simulink model "FMS"  (R2018b)
settings: configuration reference "fms_config" (kept outside this file)
values from neighbouring files (symbols this model uses):
  FMS_EXPORT = Simulink.Parameter(FMS_EXPORT_VALUE)    [fms_model_init.m]
  FMS_PARAM = Simulink.Parameter(FMS_PARAM_VALUE)    [fms_model_init.m]
undefined symbols (not defined in the file or in its folder): actuator_cmd, ax_cmd, ay_cmd, az_cmd, cmd_mask, ControlMode, ctrl_mode, DiscIntNeverNeededParam, FMS_Cmd, FMS_CONST, FMS_Error, home, mode, p_cmd, phi_cmd, PilotMode, psi_rate_cmd, q_cmd, r_cmd, reset, state, status, theta_cmd, throttle_cmd, timestamp, u_cmd, v_cmd, VehicleState, VehicleStatus, w_cmd, wp_consume, wp_current
libraries: simulink x123, FMT_Model_Lib x62, hdlsllib x13
(part 3 of 7)

== system FMS/FMS Commander/Commander/Arm/Assist/Stabilize/Heading Command/Controller ==
  motion_state : Inport
  In Bus Element : Inport  Port=2  PortName=FMS_In
  In Bus Element1 : Inport  Port=2  PortName=FMS_In
  Hold Control : Subsystem  TreatAsAtomicUnit=on
  Merge : Merge
  Move Control : Subsystem  TreatAsAtomicUnit=on
  Saturation : Saturate  UpperLimit=FMS_PARAM.MC_YAWRATE_LIM  LowerLimit=-FMS_PARAM.MC_YAWRATE_LIM
  Switch Case : SwitchCase  CaseConditions={MotionState.Hold, [MotionState.Brake, MotionState.Move]}  ShowDefaultCase=off
  psi_rate_cmd_radPs : Outport
  wires:
  Move Control/1(psi_rate_cmd_radPs) -> Merge/2
  Hold Control/1(psi_rate_cmd_radPs) -> Merge/1
  In Bus Element/1 -> Hold Control/1(FMS_In)
  Switch Case/2 -> Move Control/Action
  Switch Case/1 -> Hold Control/Action
  motion_state/1 -> Switch Case/1
  Saturation/1 -> psi_rate_cmd_radPs/1
  Merge/1 -> Saturation/1
  In Bus Element1/1 -> Move Control/1(FMS_In)

== system FMS/FMS Commander/Commander/Arm/Assist/Stabilize/Heading Command/Detect Movement ==
  FMS_In : Inport
  Abs : Abs
  Abs1 : Abs
  Bus Selector : BusSelector  OutputSignals=Pilot_Cmd.stick_yaw,INS_Out.r
  Compare To Constant : simulink/Logic and Bit Operations/Compare To Constant  relop=>  const=FMS_PARAM.MC_YAW_DZ  OutDataTypeStr=boolean
  Motion State : Stateflow chart  TreatAsAtomicUnit=on
  motion_state : Outport
  wires:
  FMS_In/1 -> Bus Selector/1
  Abs1/1 -> Compare To Constant/1
  Motion State/1(state) -> motion_state/1
  Compare To Constant/1 -> Motion State/1(motion_req)
  Abs/1 -> Motion State/2(speed)
  Bus Selector/1 -> Abs1/1  "<stick_yaw>"
  Bus Selector/2 -> Abs/1  "<r>"

== system FMS/FMS Commander/Commander/Arm/Auto/Mission/Mission_SubSystem/Heading Commander ==
  FMS_In : Inport
  Bus Selector : BusSelector  OutputSignals=Cmd_In.set_yaw
  Heading Control : Subsystem
  psi_err_rad : Outport
  psi_rad_cmd : Outport  Port=2
  wires:
  FMS_In/1 -> Heading Control/1(FMS_In), Bus Selector/1
  Heading Control/1(psi_rate_cmd_radPs) -> psi_rad_cmd/1
  Heading Control/2(psi_err_rad) -> psi_err_rad/1
  Bus Selector/1 -> Heading Control/2(psi_cmd_rad)  "<set_yaw>"

== system FMS/FMS Commander/Commander/Arm/Auto/Mission/Mission_SubSystem/Velocity Commander ==
  p1 : Inport
  p2 : Inport  Port=2
  p3 : Inport  Port=3
  In Bus Element3 : Inport  Port=4  PortName=FMS_In
  In Bus Element4 : Inport  Port=4  PortName=FMS_In
  In Bus Element : Inport  Port=4  PortName=FMS_In  Element=INS_Out.vn
  In Bus Element1 : Inport  Port=4  PortName=FMS_In  Element=INS_Out.ve
  In Bus Element2 : Inport  Port=4  PortName=FMS_In  Element=INS_Out.psi
  In Bus Element6 : Inport  Port=4  PortName=FMS_In  Element=Cmd_In.set_speed
  psi_err_rad : Inport  Port=5
  Abs : Abs
  Altitude Control : Subsystem
  Compare To Constant : simulink/Logic and Bit Operations/Compare To Constant  relop=<=  const=10/180*pi  OutDataTypeStr=boolean
  Compare To Zero : simulink/Logic and Bit Operations/Compare To Zero  relop===  OutDataTypeStr=boolean
  Cruise Speed : Subsystem
  Demux : Demux  Outputs=3
  Gain : Gain  Gain=FMS_PARAM.MC_L1_GAIN  OutDataTypeStr=single
  Hold Position : Subsystem
  L1 Reference WP : Subsystem
  Lateral Acceleration : Subsystem
  Lateral Acceleration To Speed : Subsystem
  Mux1 : Mux  Inputs=2
  Switch : Switch  Criteria=u2 > Threshold
  "Target Speed " : Subsystem
  ValidCounter : Subsystem
  u_cmd : Outport
  v_cmd : Outport  Port=2
  w_cmd : Outport  Port=3
  wires:
  p3/1 -> "Target Speed "/1(P3), Lateral Acceleration To Speed/2(p3), Lateral Acceleration/3(p3), L1 Reference WP/3(P3)
  In Bus Element1/1 -> Mux1/2
  Mux1/1 -> Lateral Acceleration/1(Vg)
  p2/1 -> "Target Speed "/2(P2), Lateral Acceleration To Speed/3(p2), L1 Reference WP/2(P2)
  Demux/2 -> v_cmd/1
  Demux/3 -> w_cmd/1
  Demux/1 -> u_cmd/1
  In Bus Element/1 -> Mux1/1
  L1 Reference WP/1(L1_WP) -> Lateral Acceleration/2(L1_WP)  "L1_WP"
  p1/1 -> L1 Reference WP/1(P1)
  Gain/1 -> Lateral Acceleration/4(L1), L1 Reference WP/4(L1)
  Lateral Acceleration/1(l1_a_cmd) -> Lateral Acceleration To Speed/1(l1_a)  "l1_a_cmd"
  In Bus Element2/1 -> Lateral Acceleration To Speed/4(psi)
  "Target Speed "/1(|Vg|) -> Lateral Acceleration To Speed/5(Vg)  "Vg"
  Lateral Acceleration To Speed/1(Vg_C_cmd) -> Altitude Control/2(Vg_C_cmd)
  psi_err_rad/1 -> Abs/1
  Abs/1 -> Compare To Constant/1
  In Bus Element3/1 -> Hold Position/1(FMS_In)
  Hold Position/1(vel_cmd) -> Switch/1
  Switch/1 -> Demux/1
  Altitude Control/1(vel_C_cmd) -> Switch/3
  In Bus Element4/1 -> Altitude Control/1(FMS_In)
  Compare To Constant/1 -> ValidCounter/1(in)
  ValidCounter/1(out) -> Compare To Zero/1
  Compare To Zero/1 -> Lateral Acceleration To Speed/7(rotating), "Target Speed "/4(rotating), Switch/2
  Cruise Speed/1(cruise_speed) -> Gain/1, "Target Speed "/3(cruise_speed), Lateral Acceleration To Speed/6(cruise_speed)
  In Bus Element6/1 -> Cruise Speed/1(config_speed)

== system FMS/FMS Commander/Commander/Arm/Auto/Mission/Mission_SubSystem/Way Points ==
  note: P1: path start point
      | P2: path end point
      | P3: vehicle point
  FMS_In : Inport
  Bus Selector : BusSelector  OutputSignals=INS_Out.x_R,INS_Out.y_R
  Bus Selector1 : BusSelector  OutputSignals=Cmd_In.sp_waypoint
  Bus Selector2 : BusSelector  OutputSignals=Cmd_In.cur_waypoint
  Mux : Mux  Inputs=2
  Reshape : Reshape  OutputDimensionality=Customize  OutputDimensions=[2,1]
  Reshape1 : Reshape  OutputDimensionality=Customize  OutputDimensions=[2,1]
  Reshape2 : Reshape  OutputDimensionality=Customize  OutputDimensions=[2,1]
  Selector : Selector  InputPortWidth=3  IndexOptions=Index vector (dialog)  Indices=[1 2]  OutputSizes=1
  Selector1 : Selector  InputPortWidth=3  IndexOptions=Index vector (dialog)  Indices=[1 2]  OutputSizes=1
  p1 : Outport
  p2 : Outport  Port=2
  p3 : Outport  Port=3
  wires:
  Reshape2/1 -> p3/1
  Reshape1/1 -> p1/1
  Reshape/1 -> p2/1
  Bus Selector/2 -> Mux/2  "<y_R>"
  Bus Selector/1 -> Mux/1  "<x_R>"
  Mux/1 -> Reshape2/1
  FMS_In/1 -> Bus Selector2/1, Bus Selector1/1, Bus Selector/1
  Bus Selector1/1 -> Selector/1  "<sp_waypoint>"
  Selector/1 -> Reshape/1
  Bus Selector2/1 -> Selector1/1  "<cur_waypoint>"
  Selector1/1 -> Reshape1/1

== system FMS/FMS Commander/Commander/Arm/Auto/Offboard/Acc_Command/Accel_Command ==
  FMS_In : Inport
  Bus Selector2 : BusSelector  OutputSignals=Auto_Cmd.ax_cmd,Auto_Cmd.ay_cmd,Auto_Cmd.az_cmd
  Mux1 : Mux  Inputs=3
  accel_cmd : Outport
  wires:
  Mux1/1 -> accel_cmd/1
  FMS_In/1 -> Bus Selector2/1
  Bus Selector2/2 -> Mux1/2  "<ay_cmd>"
  Bus Selector2/1 -> Mux1/1  "<ax_cmd>"
  Bus Selector2/3 -> Mux1/3  "<az_cmd>"

== system FMS/FMS Commander/Commander/Arm/Auto/Offboard/Acc_Command/Body_FRD ==
  acc_cmd_B : Inport
  acc_cmd_C : Outport
  wires:
  acc_cmd_B/1 -> acc_cmd_C/1

== system FMS/FMS Commander/Commander/Arm/Auto/Offboard/Acc_Command/Command_Mask ==
  FMS_In : Inport
  Bus Selector1 : BusSelector  OutputSignals=Auto_Cmd.cmd_mask
  Compare To Zero2 : simulink/Logic and Bit Operations/Compare To Zero  relop=>  OutDataTypeStr=boolean
  Mux : Mux  Inputs=3
  ax_cmd valid : simulink/Logic and Bit Operations/Bitwise Operator  logicop=AND  UseBitMask=on  BitMask=bin2dec('10000000000000000')  BitMaskRealWorld=Stored Integer
  ay_cmd valid : simulink/Logic and Bit Operations/Bitwise Operator  logicop=AND  UseBitMask=on  BitMask=bin2dec('100000000000000000')  BitMaskRealWorld=Stored Integer
  az_cmd valid : simulink/Logic and Bit Operations/Bitwise Operator  logicop=AND  UseBitMask=on  BitMask=bin2dec('1000000000000000000')  BitMaskRealWorld=Stored Integer
  acc_mask : Outport
  wires:
  az_cmd valid/1 -> Mux/3
  Compare To Zero2/1 -> acc_mask/1
  ax_cmd valid/1 -> Mux/1
  ay_cmd valid/1 -> Mux/2
  FMS_In/1 -> Bus Selector1/1
  Mux/1 -> Compare To Zero2/1
  Bus Selector1/1 -> az_cmd valid/1, ay_cmd valid/1, ax_cmd valid/1  "<cmd_mask>"

== system FMS/FMS Commander/Commander/Arm/Auto/Offboard/Acc_Command/Global_Local_NED ==
  psi : Inport
  acc_cmd_O : Inport  Port=2
  Multiply : Product  Multiplication=Matrix(*)
  Psi To DCM : FMT_Model_Lib/Transformation/Psi To DCM
      settings: SourceProductName=FMT Toolbox
  acc_cmd_C : Outport
  wires:
  psi/1 -> Psi To DCM/1
  Psi To DCM/1 -> Multiply/1  "M_CO"
  acc_cmd_O/1 -> Multiply/2
  Multiply/1 -> acc_cmd_C/1

== system FMS/FMS Commander/Commander/Arm/Auto/Offboard/Acc_Command/Local_FRD ==
  psi : Inport
  acc_cmd_R : Inport  Port=2
  Data Store Read : DataStoreRead  DataStoreName=home
  Multiply3 : Product  Multiplication=Matrix(*)
  Psi To DCM2 : FMT_Model_Lib/Transformation/Psi To DCM
      settings: SourceProductName=FMT Toolbox
  Selector : Selector  InputPortWidth=4  IndexOptions=Index vector (dialog)  Indices=4  OutputSizes=1
  Subtract : Sum  Inputs=+-
  acc_cmd_C : Outport
  wires:
  Psi To DCM2/1 -> Multiply3/1  "M_CR"
  Subtract/1 -> Psi To DCM2/1
  psi/1 -> Subtract/1
  acc_cmd_R/1 -> Multiply3/2
  Multiply3/1 -> acc_cmd_C/1
  Data Store Read/1 -> Selector/1
  Selector/1 -> Subtract/2

== system FMS/FMS Commander/Commander/Arm/Auto/Offboard/Command_Mask/Subsystem ==
  note: For global/local frame, if command valid either at x or y direction,
      | then both u and v command in control frame are valid.
  frame : Inport
  cmd_mask : Inport  Port=2
  Compare To Constant : simulink/Logic and Bit Operations/Compare To Constant  relop=<=  const=2  OutDataTypeStr=boolean
  Compare To Zero{1,6..8} (4 alike) : simulink/Logic and Bit Operations/Compare To Zero  relop=>  OutDataTypeStr=boolean
  Demux : Demux  Outputs=2
  Logical Operator : Logic  Operator=OR  Inputs=3  AllPortsSameDT=off  OutDataTypeStr=boolean
  Mux : Mux  Inputs=2
  Mux1 : Mux  Inputs=2
  Switch : Switch  Criteria=u2 > Threshold
  alt_z_w_cmd : simulink/Logic and Bit Operations/Bitwise Operator  logicop=AND  UseBitMask=on  BitMask=bin2dec('1001001000000000')  BitMaskRealWorld=Stored Integer
  lat_lon_cmd valid : simulink/Logic and Bit Operations/Bitwise Operator  logicop=AND  UseBitMask=on  BitMask=bin2dec('110000000000')  BitMaskRealWorld=Stored Integer
  x_u_cmd : simulink/Logic and Bit Operations/Bitwise Operator  logicop=AND  UseBitMask=on  BitMask=bin2dec('10000010000000')  BitMaskRealWorld=Stored Integer
  y_v_cmd : simulink/Logic and Bit Operations/Bitwise Operator  logicop=AND  UseBitMask=on  BitMask=bin2dec('100000100000000')  BitMaskRealWorld=Stored Integer
  u_valid : Outport
  v_valid : Outport  Port=2
  w_valid : Outport  Port=3
  wires:
  y_v_cmd/1 -> Compare To Zero7/1
  alt_z_w_cmd/1 -> Compare To Zero8/1
  cmd_mask/1 -> lat_lon_cmd valid/1, x_u_cmd/1, alt_z_w_cmd/1, y_v_cmd/1
  x_u_cmd/1 -> Compare To Zero6/1
  frame/1 -> Compare To Constant/1
  Compare To Constant/1 -> Switch/2
  Compare To Zero7/1 -> Mux1/2, Logical Operator/3
  Logical Operator/1 -> Mux/2, Mux/1
  Compare To Zero6/1 -> Mux1/1, Logical Operator/2
  Mux1/1 -> Switch/3
  Switch/1 -> Demux/1
  Demux/1 -> u_valid/1  "uvalid"
  Demux/2 -> v_valid/1  "vvalid"
  Mux/1 -> Switch/1
  Compare To Zero8/1 -> w_valid/1  "wvalid"
  lat_lon_cmd valid/1 -> Compare To Zero1/1
  Compare To Zero1/1 -> Logical Operator/1

== system FMS/FMS Commander/Commander/Arm/Auto/Offboard/Command_Mask/Subsystem1 ==
  note: For global/local frame, if command valid either at x or y direction,
      | then both u and v command in control frame are valid.
  frame : Inport
  cmd_mask : Inport  Port=2
  Compare To Constant : simulink/Logic and Bit Operations/Compare To Constant  relop=<=  const=2  OutDataTypeStr=boolean
  Compare To Zero10 : simulink/Logic and Bit Operations/Compare To Zero  relop=>  OutDataTypeStr=boolean
  Compare To Zero11 : simulink/Logic and Bit Operations/Compare To Zero  relop=>  OutDataTypeStr=boolean
  Compare To Zero9 : simulink/Logic and Bit Operations/Compare To Zero  relop=>  OutDataTypeStr=boolean
  Demux : Demux  Outputs=2
  Logical Operator : Logic  Operator=OR  AllPortsSameDT=off  OutDataTypeStr=boolean
  Mux : Mux  Inputs=2
  Mux1 : Mux  Inputs=2
  Switch : Switch  Criteria=u2 > Threshold
  ax_cmd : simulink/Logic and Bit Operations/Bitwise Operator  logicop=AND  UseBitMask=on  BitMask=bin2dec('10000000000000000')  BitMaskRealWorld=Stored Integer
  ay_cmd : simulink/Logic and Bit Operations/Bitwise Operator  logicop=AND  UseBitMask=on  BitMask=bin2dec('100000000000000000')  BitMaskRealWorld=Stored Integer
  az_cmd : simulink/Logic and Bit Operations/Bitwise Operator  logicop=AND  UseBitMask=on  BitMask=bin2dec('1000000000000000000')  BitMaskRealWorld=Stored Integer
  ax_valid : Outport
  ay_valid : Outport  Port=2
  az_valid : Outport  Port=3
  wires:
  ax_cmd/1 -> Compare To Zero9/1
  ay_cmd/1 -> Compare To Zero10/1
  Compare To Zero11/1 -> az_valid/1
  az_cmd/1 -> Compare To Zero11/1
  Mux1/1 -> Switch/3
  Mux/1 -> Switch/1
  Logical Operator/1 -> Mux/2, Mux/1
  frame/1 -> Compare To Constant/1
  Compare To Constant/1 -> Switch/2
  Compare To Zero10/1 -> Mux1/2, Logical Operator/2
  Compare To Zero9/1 -> Mux1/1, Logical Operator/1
  cmd_mask/1 -> az_cmd/1, ax_cmd/1, ay_cmd/1
  Switch/1 -> Demux/1
  Demux/1 -> ax_valid/1
  Demux/2 -> ay_valid/1

== system FMS/FMS Commander/Commander/Arm/Auto/Offboard/Heading_Command/Heading_Control ==
  FMS_In : Inport
  Bus Selector1 : BusSelector  OutputSignals=Auto_Cmd.cmd_mask
  Compare To Zero : simulink/Logic and Bit Operations/Compare To Zero  relop=>  OutDataTypeStr=boolean
  Error : Subsystem
  Gain2 : Gain  Gain=FMS_PARAM.MC_YAW_P  OutDataTypeStr=single
  Multiply2 : Product
  psi_cmd valid : simulink/Logic and Bit Operations/Bitwise Operator  logicop=AND  UseBitMask=on  BitMask=bin2dec('100000')  BitMaskRealWorld=Stored Integer
  psi_rate_cmd : Outport
  wires:
  Compare To Zero/1 -> Multiply2/2
  Multiply2/1 -> psi_rate_cmd/1
  FMS_In/1 -> Error/1(FMS_In), Bus Selector1/1
  Bus Selector1/1 -> psi_cmd valid/1  "<cmd_mask>"
  psi_cmd valid/1 -> Compare To Zero/1
  Gain2/1 -> Multiply2/1
  Error/1(psi_error) -> Gain2/1

== system FMS/FMS Commander/Commander/Arm/Auto/Offboard/Heading_Command/Psi_Rate_Command ==
  FMS_In : Inport
  Bus Selector2 : BusSelector  OutputSignals=Auto_Cmd.psi_rate_cmd,Auto_Cmd.cmd_mask
  Compare To Zero1 : simulink/Logic and Bit Operations/Compare To Zero  relop=>  OutDataTypeStr=boolean
  Multiply1 : Product
  psi_rate_cmd valid : simulink/Logic and Bit Operations/Bitwise Operator  logicop=AND  UseBitMask=on  BitMask=bin2dec('1000000')  BitMaskRealWorld=Stored Integer
  psi_rate_cmd : Outport
  wires:
  Bus Selector2/1 -> Multiply1/1  "<psi_rate_cmd>"
  Multiply1/1 -> psi_rate_cmd/1
  psi_rate_cmd valid/1 -> Compare To Zero1/1
  FMS_In/1 -> Bus Selector2/1
  Bus Selector2/2 -> psi_rate_cmd valid/1  "<cmd_mask>"
  Compare To Zero1/1 -> Multiply1/2

== system FMS/FMS Commander/Commander/Arm/Auto/Offboard/Velocity_Command/Position_Control ==
  FMS_In : Inport
  Body_FRD : Subsystem
  Bus Selector : BusSelector  OutputSignals=INS_Out.psi
  Bus Selector2 : BusSelector  OutputSignals=Auto_Cmd.frame
  Command_Mask : Subsystem
  Gain1 : Gain  Gain=FMS_PARAM.MC_XY_P  OutDataTypeStr=single
  Gain2 : Gain  Gain=FMS_PARAM.MC_Z_P  OutDataTypeStr=single
  Global_NED : Subsystem
  Index Vector : MultiPortSwitch  DataPortOrder=Zero-based contiguous  Inputs=4  zeroidx=on
  Local_FRD : Subsystem
  Local_NED : Subsystem
  Mux1 : Mux  Inputs=2
  Position_Command : Subsystem
  Position_State : Subsystem
  Selector : Selector  InputPortWidth=3  IndexOptions=Index vector (dialog)  Indices=[1 2]  OutputSizes=1
  Selector1 : Selector  InputPortWidth=3  IndexOptions=Index vector (dialog)  Indices=3  OutputSizes=1
  vel_cmd_C : Outport
  wires:
  Mux1/1 -> vel_cmd_C/1
  Selector1/1 -> Gain2/1
  Selector/1 -> Gain1/1
  Gain1/1 -> Mux1/1
  Gain2/1 -> Mux1/2
  Index Vector/1 -> Selector1/1, Selector/1
  Command_Mask/1(pos_mask) -> Local_NED/4(pos_mask), Global_NED/4(pos_mask), Local_FRD/4(pos_mask), Body_FRD/2(pos_mask)
  Body_FRD/1(pos_error_C) -> Index Vector/5
  Local_FRD/1(pos_error_C) -> Index Vector/4
  FMS_In/1 -> Position_State/1(FMS_In), Bus Selector2/1, Command_Mask/1(FMS_In), Position_Command/1(FMS_In), Bus Selector/1
  Position_Command/1(pos_cmd) -> Local_NED/3(pos_O_cmd), Global_NED/3(pos_O_cmd), Local_FRD/3(pos_R_cmd), Body_FRD/1(pos_C_cmd)
  Bus Selector2/1 -> Index Vector/1  "<frame>"
  Position_State/1(pos_est_O) -> Local_NED/2(pos_est_O), Local_FRD/2(pos_est_O), Global_NED/2(pos_est_O)
  Bus Selector/1 -> Global_NED/1(psi), Local_NED/1(psi), Local_FRD/1(psi)  "<psi>"
  Global_NED/1(pos_error_C) -> Index Vector/2
  Local_NED/1(pos_error_C) -> Index Vector/3

== system FMS/FMS Commander/Commander/Arm/Auto/Offboard/Velocity_Command/Velocity_Command ==
  FMS_In : Inport
  Body_FRD : Subsystem
  Bus Selector1 : BusSelector  OutputSignals=INS_Out.psi
  Bus Selector3 : BusSelector  OutputSignals=Auto_Cmd.frame
  Command_Mask : Subsystem
  Global_Local_NED : Subsystem
  Index Vector : MultiPortSwitch  DataPortOrder=Zero-based contiguous  Inputs=4  zeroidx=on
  Local_FRD : Subsystem
  Multiply : Product
  Velocity_Command : Subsystem
  vel_cmd_C : Outport
  wires:
  FMS_In/1 -> Bus Selector3/1, Bus Selector1/1, Velocity_Command/1(FMS_In), Command_Mask/1(FMS_In)
  Bus Selector3/1 -> Index Vector/1  "<frame>"
  Command_Mask/1(vel_mask) -> Multiply/2
  Index Vector/1 -> vel_cmd_C/1
  Global_Local_NED/1(vel_cmd_C) -> Index Vector/3, Index Vector/2
  Local_FRD/1(vel_cmd_C) -> Index Vector/4
  Body_FRD/1(vel_cmd_C) -> Index Vector/5
  Multiply/1 -> Global_Local_NED/2(vel_cmd_O), Body_FRD/1(vel_cmd_B), Local_FRD/2(vel_cmd_L)
  Bus Selector1/1 -> Local_FRD/1(psi), Global_Local_NED/1(psi)  "<psi>"
  Velocity_Command/1(vel_cmd) -> Multiply/1

== system FMS/FMS Commander/Commander/Arm/SubMode/Hold/Altitude Hold/Controller ==
  motion_state : Inport
  In Bus Element : Inport  Port=2  PortName=FMS_In
  In Bus Element1 : Inport  Port=2  PortName=FMS_In
  Brake Control : Subsystem  TreatAsAtomicUnit=on
  Hold Control : Subsystem  TreatAsAtomicUnit=on
  Merge : Merge  Inputs=3
  Move Control : Subsystem  TreatAsAtomicUnit=on
  Saturation1 : Saturate  UpperLimit=FMS_PARAM.MC_VEL_Z_LIM  LowerLimit=-FMS_PARAM.MC_VEL_Z_LIM
  Switch Case : SwitchCase  CaseConditions={MotionState.Hold, MotionState.Brake, MotionState.Move}  ShowDefaultCase=off
  w_cmd_mPs : Outport
  wires:
  Move Control/1(w_cmd_mPs) -> Merge/3
  Brake Control/1(psi_rate_cmd_radPs) -> Merge/2
  Hold Control/1(w_cmd_mPs) -> Merge/1
  In Bus Element/1 -> Hold Control/1(FMS_In)
  Switch Case/3 -> Move Control/Action
  Switch Case/2 -> Brake Control/Action
  Switch Case/1 -> Hold Control/Action
  motion_state/1 -> Switch Case/1
  Saturation1/1 -> w_cmd_mPs/1
  Merge/1 -> Saturation1/1
  In Bus Element1/1 -> Move Control/1(FMS_In)

== system FMS/FMS Commander/Commander/Arm/SubMode/Hold/Altitude Hold/Detect Movement ==
  FMS_In : Inport
  Abs : Abs
  Bus Selector : BusSelector  OutputSignals=INS_Out.vd
  Constant : Constant  Value=0  OutDataTypeStr=Inherit: Inherit via back propagation
  Motion Status : Stateflow chart  TreatAsAtomicUnit=on
  motion_state : Outport
  wires:
  FMS_In/1 -> Bus Selector/1
  Motion Status/1(state) -> motion_state/1
  Constant/1 -> Motion Status/1(motion_req)
  Abs/1 -> Motion Status/2(speed)
  Bus Selector/1 -> Abs/1  "<vd>"

== system FMS/FMS Commander/Commander/Arm/SubMode/Hold/Heading Hold/Controller ==
  motion_state : Inport
  In Bus Element : Inport  Port=2  PortName=FMS_In
  In Bus Element1 : Inport  Port=2  PortName=FMS_In
  Brake Control : Subsystem  TreatAsAtomicUnit=on
  Hold Control : Subsystem  TreatAsAtomicUnit=on
  Merge : Merge  Inputs=3
  Move Control : Subsystem  TreatAsAtomicUnit=on
  Saturation : Saturate  UpperLimit=FMS_PARAM.MC_YAWRATE_LIM  LowerLimit=-FMS_PARAM.MC_YAWRATE_LIM
  Switch Case : SwitchCase  CaseConditions={MotionState.Hold, MotionState.Brake, MotionState.Move}  ShowDefaultCase=off
  psi_rate_cmd_radPs : Outport
  wires:
  Move Control/1(psi_rate_cmd_radPs) -> Merge/3
  Brake Control/1(psi_rate_cmd_radPs) -> Merge/2
  Hold Control/1(psi_rate_cmd_radPs) -> Merge/1
  In Bus Element/1 -> Hold Control/1(FMS_In)
  Switch Case/3 -> Move Control/Action
  Switch Case/2 -> Brake Control/Action
  Switch Case/1 -> Hold Control/Action
  motion_state/1 -> Switch Case/1
  Saturation/1 -> psi_rate_cmd_radPs/1
  Merge/1 -> Saturation/1
  In Bus Element1/1 -> Move Control/1(FMS_In)

== system FMS/FMS Commander/Commander/Arm/SubMode/Hold/Heading Hold/Detect Movement ==
  FMS_In : Inport
  Abs : Abs
  Bus Selector : BusSelector  OutputSignals=INS_Out.r
  Constant : Constant  Value=0  OutDataTypeStr=Inherit: Inherit via back propagation
  Motion State : Stateflow chart  TreatAsAtomicUnit=on
  motion_state : Outport
  wires:
  FMS_In/1 -> Bus Selector/1
  Motion State/1(state) -> motion_state/1
  Constant/1 -> Motion State/1(motion_req)
  Abs/1 -> Motion State/2(speed)
  Bus Selector/1 -> Abs/1  "<r>"

== system FMS/FMS Commander/Commander/Arm/SubMode/Hold/Position Hold/Controller ==
  motion_state : Inport
  In Bus Element : Inport  Port=2  PortName=FMS_In
  In Bus Element1 : Inport  Port=2  PortName=FMS_In
  Brake Control : Subsystem  TreatAsAtomicUnit=on
  Hold Control : Subsystem  TreatAsAtomicUnit=on
  Merge : Merge  Inputs=3
  Move Control : Subsystem  TreatAsAtomicUnit=on
  Saturation1 : Saturate  UpperLimit=FMS_PARAM.MC_VEL_XY_LIM  LowerLimit=-FMS_PARAM.MC_VEL_XY_LIM
  Switch Case : SwitchCase  CaseConditions={MotionState.Hold, MotionState.Brake, MotionState.Move}  ShowDefaultCase=off
  uv_cmd_mPs : Outport
  wires:
  Move Control/1(uv_cmd_mPs) -> Merge/3
  Brake Control/1(uv_cmd_mPs) -> Merge/2
  Hold Control/1(uv_cmd_mPs) -> Merge/1
  In Bus Element/1 -> Hold Control/1(FMS_In)
  Switch Case/3 -> Move Control/Action
  Switch Case/2 -> Brake Control/Action
  Switch Case/1 -> Hold Control/Action
  motion_state/1 -> Switch Case/1
  Saturation1/1 -> uv_cmd_mPs/1
  Merge/1 -> Saturation1/1
  In Bus Element1/1 -> Move Control/1(FMS_In)

== system FMS/FMS Commander/Commander/Arm/SubMode/Hold/Position Hold/Detect Movement ==
  FMS_In : Inport
  Add : Sum
  Bus Selector1 : BusSelector  OutputSignals=INS_Out.vn,INS_Out.ve
  Constant : Constant  Value=0  OutDataTypeStr=Inherit: Inherit via back propagation
  Motion State : Stateflow chart  TreatAsAtomicUnit=on
  Sqrt : Sqrt  SaturateOnIntegerOverflow=on
  Square : Math  Operator=square  SaturateOnIntegerOverflow=on
  Square1 : Math  Operator=square  SaturateOnIntegerOverflow=on
  motion_state : Outport
  wires:
  FMS_In/1 -> Bus Selector1/1
  Add/1 -> Sqrt/1
  Square1/1 -> Add/2
  Square/1 -> Add/1
  Motion State/1(state) -> motion_state/1  "pos_ms"
  Sqrt/1 -> Motion State/2(speed)
  Bus Selector1/1 -> Square/1  "<vn>"
  Bus Selector1/2 -> Square1/1  "<ve>"
  Constant/1 -> Motion State/1(motion_req)

== system FMS/FMS Commander/Commander/Arm/SubMode/Land/Assist Land Speed/TD ==
  v : Inport
  Integrator : DiscreteIntegrator  SampleTime=-1  ICPrevOutput=DiscIntNeverNeededParam  ICPrevScaledInput=DiscIntNeverNeededParam
  Integrator1 : DiscreteIntegrator  SampleTime=-1  ICPrevOutput=DiscIntNeverNeededParam  ICPrevScaledInput=DiscIntNeverNeededParam
  Subtract : Sum  Inputs=+-
  "fhan " : Subsystem  mask{r0=9.806, h0=0.35}
      mask DialogControl ParameterGroupVar Prompt: fhan(v1,v2,r0,h0)
  v1 : Outport
  wires:
  "fhan "/1(fhan) -> Integrator/1
  Subtract/1 -> "fhan "/1(v1)
  Integrator/1 -> Integrator1/1, "fhan "/2(v2)  "v2"
  v/1 -> Subtract/2
  Integrator1/1 -> Subtract/1, v1/1

== system FMS/FMS Commander/Commander/Arm/SubMode/Land/Position Command/Position Control ==
  FMS_In : Inport
  land_xy_R : Inport  Port=2
  Bus Selector : BusSelector  OutputSignals=INS_Out.psi
  Bus_Selection : Subsystem
  Constant : Constant  Value=0  OutDataTypeStr=Inherit: Inherit via back propagation
  Gain2 : Gain  Gain=FMS_PARAM.MC_XY_P  OutDataTypeStr=single
  Multiply : Product  Multiplication=Matrix(*)
  Mux : Mux  Inputs=2
  Psi To DCM : FMT_Model_Lib/Transformation/Psi To DCM
      settings: SourceProductName=FMT Toolbox
  Selector : Selector  InputPortWidth=3  IndexOptions=Index vector (dialog)  Indices=[1 2]  OutputSizes=1
  Sum : Sum  Inputs=-+|
  uv_cmd_mPs : Outport
  wires:
  Selector/1 -> Gain2/1
  Mux/1 -> Multiply/2
  Multiply/1 -> Selector/1
  Constant/1 -> Mux/2
  FMS_In/1 -> Bus_Selection/1(FMS_In), Bus Selector/1
  land_xy_R/1 -> Sum/2  "land_xy_sp_R"
  Sum/1 -> Mux/1  "land_xy_err_R"
  Bus_Selection/1(xy_R_O_m) -> Sum/1  "land_xy_est_R"
  Bus Selector/1 -> Psi To DCM/1  "<psi>"
  Psi To DCM/1 -> Multiply/1  "M_CO"
  Gain2/1 -> uv_cmd_mPs/1

== system FMS/FMS Commander/Commander/Arm/SubMode/Return/Heading Commander/Heading Control ==
  FMS_In : Inport
  psi_cmd_rad : Inport  Port=2
  Bus Selector : BusSelector  OutputSignals=INS_Out.psi
  Delay : Delay  DelayLength=1  InitialConditionSource=Input port
      settings: InputPortMap=u0,p4
  Heading Control : Subsystem
  Sum : Sum  Inputs=|++
  Sum1 : Sum  Inputs=+-|
  Sum2 : Sum  Inputs=|+-
  TD : Subsystem
  psi_saturation : Subsystem
  psi_saturation1 : Subsystem
  psi_rate_cmd_radPs : Outport
  psi_err_rad : Outport  Port=2
  wires:
  psi_cmd_rad/1 -> Sum2/1, Sum1/1
  Heading Control/1(psi_rate_cmd_radPs) -> psi_rate_cmd_radPs/1
  FMS_In/1 -> Heading Control/1(FMS_In), Bus Selector/1
  TD/1(v1) -> Heading Control/2(psi_cmd_rad)
  Sum1/1 -> psi_saturation1/1(psi_in)
  Bus Selector/1 -> Sum1/2, Delay/2  "<psi>"
  psi_saturation1/1(psi_rad) -> psi_err_rad/1
  Delay/1 -> Sum2/2, TD/2(v0), Sum/2, Delay/1
  Sum2/1 -> psi_saturation/1(psi_in)
  psi_saturation/1(psi_rad) -> Sum/1
  Sum/1 -> TD/1(v)

== system FMS/FMS Commander/Commander/Arm/SubMode/Return/Heading Commander/Included Angle ==
  vec1 : Inport
  vec2 : Inport  Port=2
  2D Cross Product : FMT_Model_Lib/Math/2D Cross Product
      settings: SourceProductName=FMT Toolbox
  Acos : Trigonometry  Operator=acos
  Constant4 : Constant  OutDataTypeStr=single
  Demux : Demux  Outputs=2
  Demux1 : Demux  Outputs=2
  Dot Product : DotProduct  InputSameDT=on  OutDataTypeStr=Inherit: Inherit via internal rule
  Multiply : Product
  Mux : Mux  Inputs=2
  Mux1 : Mux  Inputs=2
  Sign1 : Signum
  Switch2 : Switch  Criteria=u2 ~= 0
  Vector Normalize : FMT_Model_Lib/Math/Vector Normalize
      settings: SourceProductName=FMT Toolbox
  Vector Normalize1 : FMT_Model_Lib/Math/Vector Normalize
      settings: SourceProductName=FMT Toolbox
  angle_rad : Outport
  wires:
  Switch2/1 -> Multiply/2
  Acos/1 -> Multiply/1
  Mux/1 -> Vector Normalize1/1
  vec2/1 -> Demux/1
  Constant4/1 -> Switch2/3
  Demux/1 -> Mux/2
  vec1/1 -> Demux1/1
  Multiply/1 -> angle_rad/1
  2D Cross Product/1 -> Sign1/1
  Vector Normalize/1 -> 2D Cross Product/2, Dot Product/1
  Demux/2 -> Mux/1
  Vector Normalize1/1 -> 2D Cross Product/1, Dot Product/2
  Sign1/1 -> Switch2/2, Switch2/1
  Demux1/2 -> Mux1/1
  Mux1/1 -> Vector Normalize/1
  Demux1/1 -> Mux1/2
  Dot Product/1 -> Acos/1

== system FMS/FMS Commander/Commander/Arm/SubMode/Return/Velocity Commander/Altitude Control ==
  FMS_In : Inport
  Vg_C_cmd : Inport  Port=2
  Bus Selector3 : BusSelector  OutputSignals=INS_Out.h_R
  Gain : Gain  Gain=FMS_PARAM.MC_Z_P
  Mux : Mux  Inputs=2
  Saturation1 : Saturate  UpperLimit=FMS_PARAM.MC_VEL_Z_LIM  LowerLimit=-FMS_PARAM.MC_VEL_Z_LIM
  Selector : Selector  InputPortWidth=3  IndexOptions=Index vector (dialog)  Indices=[1 2]  OutputSizes=1
  Sum2 : Sum  Inputs=|+-
  Target Height : Subsystem
  vel_C_cmd : Outport
  wires:
  FMS_In/1 -> Bus Selector3/1, Target Height/1(FMS_In)
  Bus Selector3/1 -> Sum2/1  "<h_R>"
  Sum2/1 -> Gain/1
  Gain/1 -> Saturation1/1
  Target Height/1(h_R_sp) -> Sum2/2  "h_R_sp"
  Vg_C_cmd/1 -> Selector/1
  Selector/1 -> Mux/1
  Saturation1/1 -> Mux/2
  Mux/1 -> vel_C_cmd/1

== system FMS/FMS Commander/Commander/Arm/SubMode/Return/Velocity Commander/Cruise Speed ==
  config_speed : Inport
  Compare To Zero : simulink/Logic and Bit Operations/Compare To Zero  relop=>  OutDataTypeStr=boolean
  Switch2 : Switch  Criteria=u2 > Threshold
  vel : Constant  Value=FMS_PARAM.MC_CRUISE_SPEED  OutDataTypeStr=single
  cruise_speed : Outport
  wires:
  config_speed/1 -> Compare To Zero/1, Switch2/1
  Compare To Zero/1 -> Switch2/2
  vel/1 -> Switch2/3  "|Vg|"
  Switch2/1 -> cruise_speed/1

== system FMS/FMS Commander/Commander/Arm/SubMode/Return/Velocity Commander/Hold Position ==
  FMS_In : Inport
  Altitude Hold : Subsystem
  Mux : Mux  Inputs=3
  Position Hold : Subsystem
  vel_cmd : Outport
  wires:
  FMS_In/1 -> Altitude Hold/1(FMS_In), Position Hold/1(FMS_In)
  Position Hold/2(v_cmd_mPs) -> Mux/2
  Altitude Hold/1(w_cmd_mPs) -> Mux/3
  Position Hold/1(u_cmd_mPs) -> Mux/1
  Mux/1 -> vel_cmd/1

== system FMS/FMS Commander/Commander/Arm/SubMode/Return/Velocity Commander/L1 Reference WP ==
  P1 : Inport
  P2 : Inport  Port=2
  P3 : Inport  Port=3
  L1 : Inport  Port=4
  Compare To Constant : simulink/Logic and Bit Operations/Compare To Constant  relop=>=  const=0  OutDataTypeStr=boolean
  Compare To Constant1 : simulink/Logic and Bit Operations/Compare To Constant  relop=>  const=0  OutDataTypeStr=boolean
  NearbyRefWP : MATLAB Function  TreatAsAtomicUnit=on
  OutRegionRegWP : MATLAB Function  TreatAsAtomicUnit=on
  Reshape : Reshape  OutputDimensionality=Customize  OutputDimensions=[2,1]
  SearchL1RefWP : MATLAB Function  TreatAsAtomicUnit=on
  Switch : Switch  Criteria=u2 > Threshold
  Switch1 : Switch  Criteria=u2 > Threshold
  L1_WP : Outport
  wires:
  Reshape/1 -> L1_WP/1
  Compare To Constant/1 -> Switch/2
  NearbyRefWP/2(d) -> Compare To Constant1/1  "distance"
  SearchL1RefWP/2(u) -> Compare To Constant/1  "l1_u"
  Compare To Constant1/1 -> Switch1/2
  P1/1 -> SearchL1RefWP/1(P1), OutRegionRegWP/1(P1)
  P2/1 -> SearchL1RefWP/2(P2), NearbyRefWP/1(P2), OutRegionRegWP/2(P2)
  P3/1 -> NearbyRefWP/2(P3), SearchL1RefWP/3(P3), OutRegionRegWP/3(P3)
  Switch/1 -> Switch1/3
  L1/1 -> SearchL1RefWP/4(L1), NearbyRefWP/3(L1)
  OutRegionRegWP/1(P) -> Switch/3  "out_WP"
  Switch1/1 -> Reshape/1
  SearchL1RefWP/1(P) -> Switch/1  "L1_Ref_P"
  NearbyRefWP/1(P) -> Switch1/1  "NearbyWP"

== system FMS/FMS Commander/Commander/Arm/SubMode/Return/Velocity Commander/Lateral Acceleration ==
  Vg : Inport
  L1_WP : Inport  Port=2
  p3 : Inport  Port=3
  L1 : Inport  Port=4
  Constant : Constant  Value=0.5  OutDataTypeStr=Inherit: Inherit via back propagation
  Divide : Product  Inputs=*/
  Gain : Gain  Gain=2
  Included Angle : Subsystem
  Max : MinMax  Function=max  Inputs=2
  Min : MinMax  Inputs=2
  Multiply1 : Product
  Saturation : Saturate  UpperLimit=pi/2  LowerLimit=-pi/2
  Sin : Trigonometry
  Square : Math  Operator=square  SaturateOnIntegerOverflow=on
  Subtract : Sum  Inputs=+-
  Vector Modulus : FMT_Model_Lib/Math/Vector Modulus
      settings: SourceProductName=FMT Toolbox
  Vector Modulus1 : FMT_Model_Lib/Math/Vector Modulus
      settings: SourceProductName=FMT Toolbox
  Vector Normalize : FMT_Model_Lib/Math/Vector Normalize
      settings: SourceProductName=FMT Toolbox
  Vector Normalize1 : FMT_Model_Lib/Math/Vector Normalize
      settings: SourceProductName=FMT Toolbox
  l1_a_cmd : Outport
  wires:
  Saturation/1 -> Sin/1
  Included Angle/1(angle_rad) -> Saturation/1  "L1_alpha"
  Vector Modulus/1 -> Square/1
  Subtract/1 -> Vector Modulus1/1, Vector Normalize1/1
  Gain/1 -> Multiply1/2
  L1_WP/1 -> Subtract/1
  Vector Normalize/1 -> Included Angle/1(vec1)
  Multiply1/1 -> Divide/1
  Divide/1 -> l1_a_cmd/1  "l1_a_cmd"
  Vector Normalize1/1 -> Included Angle/2(vec2)
  Square/1 -> Gain/1
  L1/1 -> Min/1
  Vg/1 -> Vector Normalize/1, Vector Modulus/1
  Sin/1 -> Multiply1/1  "sin_alpha"
  p3/1 -> Subtract/2
  Vector Modulus1/1 -> Max/1
  Constant/1 -> Max/2
  Max/1 -> Min/2
  Min/1 -> Divide/2

== system FMS/FMS Commander/Commander/Arm/SubMode/Return/Velocity Commander/Lateral Acceleration To Speed ==
  note: If included angle between initial p3p2 and current p3p2 is larger
      | than pi/2, we need reset initial p3p2 and l1_psi
  l1_a : Inport
  p3 : Inport  Port=2
  p2 : Inport  Port=3
  psi : Inport  Port=4
  Vg : Inport  Port=5
  cruise_speed : Inport  Port=6
  rotating : Inport  Port=7
  Abs : Abs
  Compare To Constant : simulink/Logic and Bit Operations/Compare To Constant  relop=>  const=pi/2  OutDataTypeStr=boolean
  Constant1 : Constant  Value=0.5  OutDataTypeStr=single
  Delay : Delay  DelayLength=1  InitialConditionSource=Input port  ExternalReset=Level
      settings: InputPortMap=u0,r5,p4
  Delay1 : Delay  DelayLength=1
  Divide1 : Product  Inputs=*/
  Ground Speed : Subsystem
  Included Angle : Subsystem
  Logical Operator : Logic  Operator=OR  AllPortsSameDT=off  OutDataTypeStr=boolean
  Multiply : Product  Multiplication=Matrix(*)
  Rotation Matrix : Subsystem
  Saturation : Saturate  UpperLimit=pi/10  LowerLimit=-pi/10
  Saturation Dynamic : simulink/Discontinuities/Saturation Dynamic  OutMin=[]  OutMax=[]  OutDataTypeStr=Inherit: Same as second input  OutDataType=fixdt(1, 16)  OutScaling=2^-10  DoSatur=off
  Sum : Sum  Inputs=|+-
  Sum1 : Sum  Inputs=+-|
  Vg_C_cmd : Outport
  wires:
  psi/1 -> Rotation Matrix/2(psi)
  Sum/1 -> Included Angle/1(vec1), Ground Speed/2(p3p2)
  l1_a/1 -> Divide1/1
  Vg/1 -> Ground Speed/1(Vg), Saturation Dynamic/2
  p3/1 -> Sum1/2, Delay/3
  Multiply/1 -> Vg_C_cmd/1
  Rotation Matrix/1(M_CO) -> Multiply/1
  Divide1/1 -> Saturation/1
  Ground Speed/1(Vg_O_cmd) -> Multiply/2  "Vg_O_cmd"
  Delay/1 -> Delay/1, Sum/2
  Saturation/1 -> Rotation Matrix/1(l1_omega)
  cruise_speed/1 -> Saturation Dynamic/1
  Sum1/1 -> Included Angle/2(vec2)
  Included Angle/1(angle_rad) -> Abs/1
  Abs/1 -> Compare To Constant/1
  rotating/1 -> Logical Operator/1
  Compare To Constant/1 -> Delay1/1
  Logical Operator/1 -> Delay/2, Rotation Matrix/3(reset)
  p2/1 -> Sum/1, Sum1/1
  Delay1/1 -> Logical Operator/2
  Saturation Dynamic/1 -> Divide1/2
  Constant1/1 -> Saturation Dynamic/3

== system FMS/FMS Commander/Commander/Arm/SubMode/Return/Velocity Commander/Target Speed  ==
  P3 : Inport
  P2 : Inport  Port=2
  cruise_speed : Inport  Port=3
  rotating : Inport  Port=4
  Acceleration_Speed : DiscreteIntegrator  ExternalReset=level  SampleTime=-1  UpperSaturationLimit=FMS_PARAM.CRUISE_SPEED  LowerSaturationLimit=0  ICPrevOutput=DiscIntNeverNeededParam  ICPrevScaledInput=DiscIntNeverNeededParam
  Constant : Constant  Value=FMS_PARAM.MC_CRUISE_ACC  OutDataTypeStr=single
  Constant1 : Constant  Value=0.5  OutDataTypeStr=single
  Constant2 : Constant  Value=0  OutDataTypeStr=single
  Gain : Gain  Gain=0.5  OutDataTypeStr=Inherit: Same as input
  L1_GAIN : Gain  Gain=FMS_PARAM.MC_L1_GAIN  OutDataTypeStr=single
  Saturation Dynamic : simulink/Discontinuities/Saturation Dynamic  OutMin=[]  OutMax=[]  OutDataTypeStr=Inherit: Same as second input  OutDataType=fixdt(1, 16)  OutScaling=2^-10  DoSatur=off
  Saturation Dynamic1 : simulink/Discontinuities/Saturation Dynamic  OutMin=[]  OutMax=[]  OutDataTypeStr=Inherit: Same as second input  OutDataType=fixdt(1, 16)  OutScaling=2^-10  DoSatur=off
  Sum : Sum  Inputs=|+-
  Sum1 : Sum  Inputs=-+|
  Sum2 : Sum  Inputs=-+|
  Switch : Switch
  Switch1 : Switch
  Vector Modulus : FMT_Model_Lib/Math/Vector Modulus
      settings: SourceProductName=FMT Toolbox
  Vg : Outport
  wires:
  Gain/1 -> Saturation Dynamic/2
  Switch/1 -> Sum1/1, Switch1/1
  Vector Modulus/1 -> Sum2/2, Gain/1
  Sum/1 -> Vector Modulus/1
  P2/1 -> Sum/2
  P3/1 -> Sum/1
  Saturation Dynamic/1 -> Switch/3
  Constant/1 -> Acceleration_Speed/1
  Saturation Dynamic1/1 -> Switch1/3, Sum1/2
  Sum1/1 -> Switch1/2
  Switch1/1 -> Vg/1
  rotating/1 -> Acceleration_Speed/2
  cruise_speed/1 -> L1_GAIN/1, Saturation Dynamic1/1, Saturation Dynamic/1, Switch/1
  Constant1/1 -> Saturation Dynamic/3
  Acceleration_Speed/1 -> Saturation Dynamic1/2
  Constant2/1 -> Saturation Dynamic1/3
  L1_GAIN/1 -> Sum2/1
  Sum2/1 -> Switch/2

== system FMS/FMS Commander/Commander/Arm/SubMode/Return/Velocity Commander/ValidCounter ==
  in : Inport
  Compare To Constant : simulink/Logic and Bit Operations/Compare To Constant  relop=>  const=3.0  OutDataTypeStr=boolean
  Discrete-Time Integrator : DiscreteIntegrator  IntegratorMethod=Accumulation: Forward Euler  SampleTime=-1  LimitOutput=on  UpperSaturationLimit=100  LowerSaturationLimit=0  ICPrevOutput=DiscIntNeverNeededParam  ICPrevScaledInput=DiscIntNeverNeededParam
  out : Outport
  wires:
  in/1 -> Discrete-Time Integrator/1
  Discrete-Time Integrator/1 -> Compare To Constant/1
  Compare To Constant/1 -> out/1

== system FMS/FMS Commander/Commander/Arm/SubMode/Takeoff/Climb Speed/TD ==
  v : Inport
  Integrator : DiscreteIntegrator  SampleTime=-1  ICPrevOutput=DiscIntNeverNeededParam  ICPrevScaledInput=DiscIntNeverNeededParam
  Integrator1 : DiscreteIntegrator  SampleTime=-1  ICPrevOutput=DiscIntNeverNeededParam  ICPrevScaledInput=DiscIntNeverNeededParam
  Subtract : Sum  Inputs=+-
  "fhan " : Subsystem  mask{r0=9.806, h0=0.35}
      mask DialogControl ParameterGroupVar Prompt: fhan(v1,v2,r0,h0)
  v1 : Outport
  wires:
  "fhan "/1(fhan) -> Integrator/1
  Subtract/1 -> "fhan "/1(v1)
  Integrator/1 -> Integrator1/1, "fhan "/2(v2)  "v2"
  v/1 -> Subtract/2
  Integrator1/1 -> Subtract/1, v1/1

== system FMS/FMS Commander/Commander/Arm/SubMode/Takeoff/Track Position/Bus_Selection ==
  FMS_In : Inport
  Bus Selector2 : BusSelector  OutputSignals=INS_Out.x_R,INS_Out.y_R
  Mux : Mux  Inputs=2
  xy_est_R : Outport
  wires:
  Bus Selector2/2 -> Mux/2  "<y_R>"
  Mux/1 -> xy_est_R/1
  Bus Selector2/1 -> Mux/1  "<x_R>"
  FMS_In/1 -> Bus Selector2/1

== system FMS/FMS Commander/Commander/Arm/SubMode/Takeoff/Track Position/Target Position ==
  FMS_In : Inport
  Bus Selector1 : BusSelector  OutputSignals=Cmd_In.sp_waypoint
  Bus Selector2 : BusSelector  OutputSignals=INS_Out.x_R,INS_Out.y_R,INS_Out.h_R
  Divide : Product  Inputs=/*
  Multiply : Product
  Mux : Mux  Inputs=3
  Reshape : Reshape  OutputDimensionality=Column vector (2-D)  OutputDimensions=[2,1]
  Saturation : Saturate  UpperLimit=1  LowerLimit=0
  Selector1 : Selector  InputPortWidth=3  IndexOptions=Index vector (dialog)  Indices=[1 2]  OutputSizes=1
  Selector2 : Selector  InputPortWidth=3  IndexOptions=Index vector (dialog)  Indices=3  OutputSizes=1
  Selector3 : Selector  InputPortWidth=3  IndexOptions=Index vector (dialog)  Indices=3  OutputSizes=1
  Selector4 : Selector  InputPortWidth=3  IndexOptions=Index vector (dialog)  Indices=[1 2]  OutputSizes=1
  Sum1 : Sum  Inputs=|+-
  Sum2 : Sum  Inputs=-+|
  Sum3 : Sum  Inputs=|+-
  Sum4 : Sum  Inputs=|++
  cur_waypoint : Delay  DelayLength=1  InitialConditionSource=Input port  InitialCondition=single([0 0])
      settings: InputPortMap=u0,p4
  xy_cmd_R : Outport
  wires:
  Bus Selector2/3 -> Mux/3, Sum2/2  "<h_R>"
  Saturation/1 -> Multiply/2
  Selector3/1 -> Sum2/1, Sum1/2
  cur_waypoint/1 -> Selector3/1, Selector4/1, cur_waypoint/1
  Sum2/1 -> Divide/2
  Selector2/1 -> Sum1/1
  Divide/1 -> Saturation/1
  FMS_In/1 -> Bus Selector2/1, Bus Selector1/1
  Sum1/1 -> Divide/1
  Bus Selector1/1 -> Selector1/1, Selector2/1  "<sp_waypoint>"
  Selector1/1 -> Sum3/1
  Selector4/1 -> Sum4/2, Sum3/2
  Sum3/1 -> Multiply/1
  Multiply/1 -> Sum4/1
  Sum4/1 -> Reshape/1
  Reshape/1 -> xy_cmd_R/1
  Mux/1 -> cur_waypoint/2
  Bus Selector2/2 -> Mux/2  "<y_R>"
  Bus Selector2/1 -> Mux/1  "<x_R>"

== system FMS/FMS Commander/Commander/Arm/Assist/Altitude/Altitude Command/Controller/Hold Control ==
  FMS_In : Inport
  Action Port : ActionPort  InitializeStates=reset  ActionType=case
  Bus_Selection : Subsystem
  Delay : Delay  DelayLength=1  InitialConditionSource=Input port
      settings: InputPortMap=u0,p4
  Gain2 : Gain  Gain=FMS_PARAM.MC_Z_P  OutDataTypeStr=single
  Sum : Sum  Inputs=-+|
  w_cmd_mPs : Outport
  wires:
  FMS_In/1 -> Bus_Selection/1(FMS_In)
  Delay/1 -> Sum/2, Delay/1  "z_cmd_R"
  Sum/1 -> Gain2/1  "z_err_R"
  Bus_Selection/1(z_R_m) -> Delay/2, Sum/1  "z_est_R"
  Gain2/1 -> w_cmd_mPs/1

== system FMS/FMS Commander/Commander/Arm/Assist/Altitude/Altitude Command/Controller/Move Control ==
  FMS_In : Inport
  Action Port : ActionPort  InitializeStates=reset  ActionType=case
  Assist Land Speed : Subsystem
  Bus Selector : BusSelector  OutputSignals=Pilot_Cmd.stick_throttle
  Bus Selector1 : BusSelector  OutputSignals=INS_Out.flag,INS_Out.h_AGL
  Compare To Constant : simulink/Logic and Bit Operations/Compare To Constant  relop=<=  const=FMS_PARAM.MC_ASSIST_LAND_H  OutDataTypeStr=boolean
  Compare To Constant1 : simulink/Logic and Bit Operations/Compare To Constant  relop=>  const=0  OutDataTypeStr=boolean
  DeadZone : Subsystem  mask{th=FMS_PARAM.MC_THROTTLE_DZ}
      mask prompts: th "Threshold"
      mask Display: disp('Dead Zone')
  Gain1 : Gain  Gain=-FMS_PARAM.MC_VEL_Z_LIM  OutDataTypeStr=single
  Logical Operator : Logic  Inputs=3  AllPortsSameDT=off  OutDataTypeStr=boolean
  Switch : Switch  Criteria=u2 > Threshold
  cmd_p valid : simulink/Logic and Bit Operations/Bitwise Operator  logicop=AND  UseBitMask=on  BitMask=bin2dec('100000000')  BitMaskRealWorld=Stored Integer
  w_cmd_mPs : Outport
  wires:
  cmd_p valid/1 -> Logical Operator/2  "h_AGL_valid"
  Compare To Constant1/1 -> Logical Operator/1
  Bus Selector1/1 -> cmd_p valid/1  "<flag>"
  Compare To Constant/1 -> Logical Operator/3
  DeadZone/1(y) -> Gain1/1
  Bus Selector1/2 -> Compare To Constant/1  "<h_AGL>"
  Bus Selector/1 -> DeadZone/1(u)  "<stick_throttle>"
  Logical Operator/1 -> Switch/2
  Gain1/1 -> Compare To Constant1/1, Assist Land Speed/1(u), Switch/3
  FMS_In/1 -> Bus Selector1/1, Bus Selector/1
  Assist Land Speed/1(y) -> Switch/1
  Switch/1 -> w_cmd_mPs/1

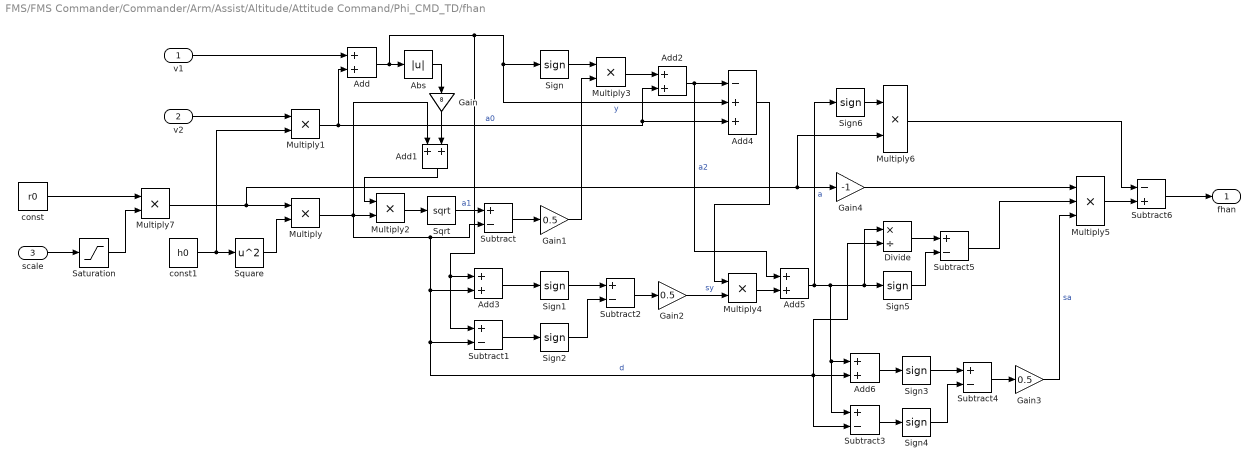
== system FMS/FMS Commander/Commander/Arm/Assist/Altitude/Attitude Command/Phi_CMD_TD/fhan  ==
  v1 : Inport
  v2 : Inport  Port=2
  scale : Inport  Port=3
  Abs : Abs
  Add{,1..3,5..6} (6 alike) : Sum  OutDataTypeStr=Inherit: Same as first input
  Add4 : Sum  Inputs=-++
  Divide : Product  Inputs=*/
  Gain : Gain  Gain=8
  Gain1 : Gain  Gain=0.5  OutDataTypeStr=Inherit: Same as input
  Gain2 : Gain  Gain=0.5  OutDataTypeStr=Inherit: Same as input
  Gain3 : Gain  Gain=0.5  OutDataTypeStr=Inherit: Same as input
  Gain4 : Gain  Gain=-1  OutDataTypeStr=Inherit: Same as input
  Multiply{,1..3} (4 alike) : Product  OutDataTypeStr=Inherit: Same as first input
  Multiply4 : Product  OutDataTypeStr=single
  Multiply5 : Product  Inputs=3
  Multiply6 : Product  OutDataTypeStr=single
  Multiply7 : Product
  Saturation : Saturate  UpperLimit=1  LowerLimit=0
  Sign{,1..6} (7 alike) : Signum
  Sqrt : Sqrt  SaturateOnIntegerOverflow=on
  Square : Math  Operator=square  SaturateOnIntegerOverflow=on
  Subtract{,1..5} (6 alike) : Sum  Inputs=+-  OutDataTypeStr=Inherit: Same as first input
  Subtract6 : Sum  Inputs=-+  OutDataTypeStr=Inherit: Same as first input
  const : Constant  Value=r0  OutDataTypeStr=single
  const1 : Constant  Value=h0  OutDataTypeStr=single
  fhan : Outport
  wires:
  v1/1 -> Add/1
  Sign/1 -> Multiply3/1
  Gain2/1 -> Multiply4/2  "sy"
  v2/1 -> Multiply1/1
  Gain3/1 -> Multiply5/3  "sa"
  Subtract/1 -> Gain1/1
  Subtract6/1 -> fhan/1
  Sign2/1 -> Subtract2/2
  Sign4/1 -> Subtract4/2
  Abs/1 -> Gain/1
  Add4/1 -> Multiply4/1
  Sign5/1 -> Subtract5/2
  Sqrt/1 -> Subtract/1  "a1"
  Subtract3/1 -> Sign4/1
  Add1/1 -> Multiply2/1
  Subtract1/1 -> Sign2/1
  Divide/1 -> Subtract5/1
  Multiply3/1 -> Add2/1
  Gain/1 -> Add1/2
  Multiply7/1 -> Multiply6/2, Gain4/1, Multiply/1
  Add3/1 -> Sign1/1
  Subtract5/1 -> Multiply5/2
  Multiply4/1 -> Add5/2
  const1/1 -> Multiply1/2, Square/1
  Add5/1 -> Sign6/1, Sign5/1, Divide/1, Subtract3/1, Add6/1  "a"
  Multiply1/1 -> Add4/3, Add2/2, Add/2  "a0"
  Add/1 -> Subtract1/1, Add3/1, Add4/2, Sign/1, Abs/1  "y"
  Subtract2/1 -> Gain2/1
  Add2/1 -> Add4/1, Add5/1  "a2"
  Subtract4/1 -> Gain3/1
  Gain4/1 -> Multiply5/1
  Multiply5/1 -> Subtract6/2
  Sign6/1 -> Multiply6/1
  Sign3/1 -> Subtract4/1
  Add6/1 -> Sign3/1
  Multiply/1 -> Subtract/2, Divide/2, Subtract3/2, Add6/2, Subtract1/2, Add3/2, Add1/1, Multiply2/2  "d"
  Multiply6/1 -> Subtract6/1
  Gain1/1 -> Multiply3/2
  Square/1 -> Multiply/2
  Multiply2/1 -> Sqrt/1
  Sign1/1 -> Subtract2/1
  scale/1 -> Saturation/1
  const/1 -> Multiply7/1
  Saturation/1 -> Multiply7/2

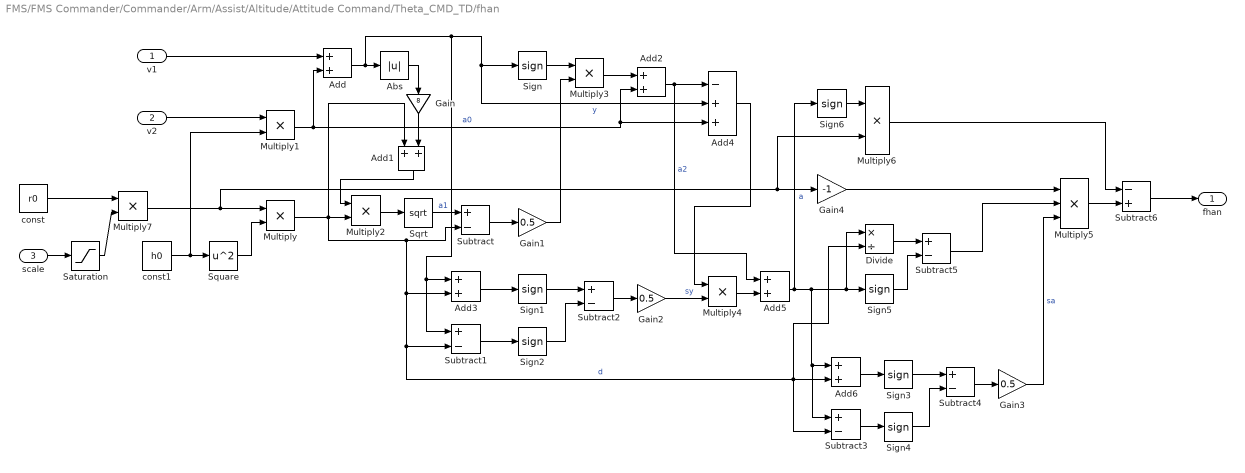
== system FMS/FMS Commander/Commander/Arm/Assist/Altitude/Attitude Command/Theta_CMD_TD/fhan  ==
  v1 : Inport
  v2 : Inport  Port=2
  scale : Inport  Port=3
  Abs : Abs
  Add{,1..3,5..6} (6 alike) : Sum  OutDataTypeStr=Inherit: Same as first input
  Add4 : Sum  Inputs=-++
  Divide : Product  Inputs=*/
  Gain : Gain  Gain=8
  Gain1 : Gain  Gain=0.5  OutDataTypeStr=Inherit: Same as input
  Gain2 : Gain  Gain=0.5  OutDataTypeStr=Inherit: Same as input
  Gain3 : Gain  Gain=0.5  OutDataTypeStr=Inherit: Same as input
  Gain4 : Gain  Gain=-1  OutDataTypeStr=Inherit: Same as input
  Multiply{,1..3} (4 alike) : Product  OutDataTypeStr=Inherit: Same as first input
  Multiply4 : Product  OutDataTypeStr=single
  Multiply5 : Product  Inputs=3
  Multiply6 : Product  OutDataTypeStr=single
  Multiply7 : Product
  Saturation : Saturate  UpperLimit=1  LowerLimit=0
  Sign{,1..6} (7 alike) : Signum
  Sqrt : Sqrt  SaturateOnIntegerOverflow=on
  Square : Math  Operator=square  SaturateOnIntegerOverflow=on
  Subtract{,1..5} (6 alike) : Sum  Inputs=+-  OutDataTypeStr=Inherit: Same as first input
  Subtract6 : Sum  Inputs=-+  OutDataTypeStr=Inherit: Same as first input
  const : Constant  Value=r0  OutDataTypeStr=single
  const1 : Constant  Value=h0  OutDataTypeStr=single
  fhan : Outport
  wires:
  v1/1 -> Add/1
  Sign/1 -> Multiply3/1
  Gain2/1 -> Multiply4/2  "sy"
  v2/1 -> Multiply1/1
  Gain3/1 -> Multiply5/3  "sa"
  Subtract/1 -> Gain1/1
  Subtract6/1 -> fhan/1
  Sign2/1 -> Subtract2/2
  Sign4/1 -> Subtract4/2
  Abs/1 -> Gain/1
  Add4/1 -> Multiply4/1
  Sign5/1 -> Subtract5/2
  Sqrt/1 -> Subtract/1  "a1"
  Subtract3/1 -> Sign4/1
  Add1/1 -> Multiply2/1
  Subtract1/1 -> Sign2/1
  Divide/1 -> Subtract5/1
  Multiply3/1 -> Add2/1
  Gain/1 -> Add1/2
  Multiply7/1 -> Multiply6/2, Gain4/1, Multiply/1
  Add3/1 -> Sign1/1
  Subtract5/1 -> Multiply5/2
  Multiply4/1 -> Add5/2
  const1/1 -> Multiply1/2, Square/1
  Add5/1 -> Sign6/1, Sign5/1, Divide/1, Subtract3/1, Add6/1  "a"
  Multiply1/1 -> Add4/3, Add2/2, Add/2  "a0"
  Add/1 -> Subtract1/1, Add3/1, Add4/2, Sign/1, Abs/1  "y"
  Subtract2/1 -> Gain2/1
  Add2/1 -> Add4/1, Add5/1  "a2"
  Subtract4/1 -> Gain3/1
  Gain4/1 -> Multiply5/1
  Multiply5/1 -> Subtract6/2
  Sign6/1 -> Multiply6/1
  Sign3/1 -> Subtract4/1
  Add6/1 -> Sign3/1
  Multiply/1 -> Subtract/2, Divide/2, Subtract3/2, Add6/2, Subtract1/2, Add3/2, Add1/1, Multiply2/2  "d"
  Multiply6/1 -> Subtract6/1
  Gain1/1 -> Multiply3/2
  Square/1 -> Multiply/2
  Multiply2/1 -> Sqrt/1
  Sign1/1 -> Subtract2/1
  scale/1 -> Saturation/1
  Saturation/1 -> Multiply7/2
  const/1 -> Multiply7/1

== system FMS/FMS Commander/Commander/Arm/Assist/Altitude/Heading Command/Controller/Hold Control ==
  FMS_In : Inport
  Action Port : ActionPort  InitializeStates=reset  ActionType=case
  Bus_Selection : Subsystem
  Delay : Delay  DelayLength=1  InitialConditionSource=Input port
      settings: InputPortMap=u0,p4
  Gain2 : Gain  Gain=FMS_PARAM.MC_YAW_P  OutDataTypeStr=single
  Sum : Sum  Inputs=-+|
  psi_err_saturation : Subsystem
  psi_rate_cmd_radPs : Outport
  wires:
  Gain2/1 -> psi_rate_cmd_radPs/1
  FMS_In/1 -> Bus_Selection/1(FMS_In)
  Delay/1 -> Sum/2, Delay/1  "psi_cmd_rad"
  Sum/1 -> psi_err_saturation/1(psi_err_in)  "psi_error_rad"
  psi_err_saturation/1(psi_err_rad) -> Gain2/1
  Bus_Selection/1(psi_rad) -> Delay/2, Sum/1  "psi_est_rad"

== system FMS/FMS Commander/Commander/Arm/Assist/Altitude/Heading Command/Controller/Move Control ==
  FMS_In : Inport
  Action Port : ActionPort  InitializeStates=reset  ActionType=case
  Bus Selector : BusSelector  OutputSignals=Pilot_Cmd.stick_yaw
  DeadZone : Subsystem  mask{th=FMS_PARAM.MC_YAW_DZ}
      mask prompts: th "Threshold"
      mask Display: disp('Dead Zone')
  Gain1 : Gain  Gain=FMS_PARAM.MC_YAWRATE_LIM  OutDataTypeStr=single
  TD : Subsystem
  psi_rate_cmd_radPs : Outport
  wires:
  TD/1(v1) -> psi_rate_cmd_radPs/1
  FMS_In/1 -> Bus Selector/1
  Bus Selector/1 -> DeadZone/1(u)  "<stick_yaw>"
  DeadZone/1(y) -> Gain1/1
  Gain1/1 -> TD/1(v)

== system FMS/FMS Commander/Commander/Arm/Assist/Position/Altitude Command/Controller/Hold Control ==
  FMS_In : Inport
  Action Port : ActionPort  InitializeStates=reset  ActionType=case
  Bus_Selection : Subsystem
  Delay : Delay  DelayLength=1  InitialConditionSource=Input port
      settings: InputPortMap=u0,p4
  Gain2 : Gain  Gain=FMS_PARAM.MC_Z_P  OutDataTypeStr=single
  Sum : Sum  Inputs=-+|
  w_cmd_mPs : Outport
  wires:
  FMS_In/1 -> Bus_Selection/1(FMS_In)
  Delay/1 -> Sum/2, Delay/1  "z_cmd_R"
  Sum/1 -> Gain2/1  "z_err_R"
  Bus_Selection/1(z_R_m) -> Delay/2, Sum/1  "z_est_R"
  Gain2/1 -> w_cmd_mPs/1
